simulink model "two"  (R2026a)
settings: Solver=VariableStepAuto
values from neighbouring files (symbols this model uses):
  L = 0.5    [MATLAB_6b.m]    (also in lab6_c.m)
  r = 0.1    [MATLAB_6b.m]    (also in lab6_c.m)
  WL = (V/r)-((L*Yr)/(2*r))    (= 20)    [MATLAB_6b.m]
  WR = (V/r)+((L*Yr)/(2*r))    (= 20)    [MATLAB_6b.m]
settings Model: Creator=m282256  LastModifiedBy=m282256

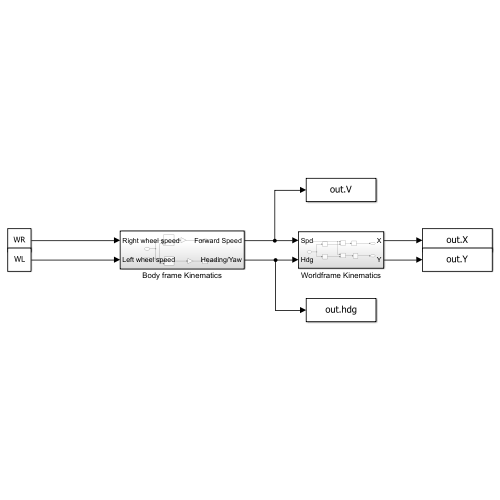
[thumbnail: Simulink's stored preview of the top-level diagram]
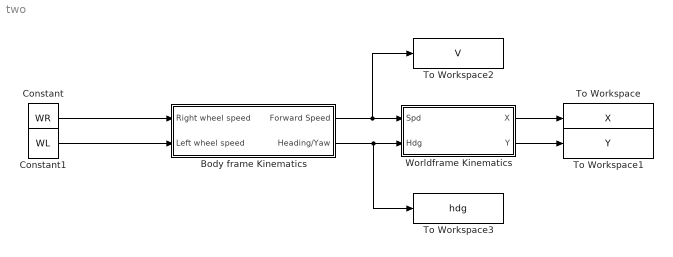
== system two ==
  Body frame Kinematics : Subsystem
  Constant : Constant  Value=WR
  Constant1 : Constant  Value=WL
  To Workspace : ToWorkspace  VariableName=X  SaveFormat=Timeseries  SampleTime=-1
  To Workspace1 : ToWorkspace  VariableName=Y  SaveFormat=Timeseries  SampleTime=-1
  To Workspace2 : ToWorkspace  VariableName=V  SaveFormat=Timeseries  SampleTime=-1
  To Workspace3 : ToWorkspace  VariableName=hdg  SaveFormat=Timeseries  SampleTime=-1
  Worldframe Kinematics : Subsystem
  wires:
  Constant1/1 -> Body frame Kinematics/2(Left wheel speed)
  Constant/1 -> Body frame Kinematics/1(Right wheel speed)
  Body frame Kinematics/2(Heading/Yaw) -> To Workspace3/1, Worldframe Kinematics/2(Hdg)
  Body frame Kinematics/1(Forward Speed) -> To Workspace2/1, Worldframe Kinematics/1(Spd)
  Worldframe Kinematics/2(Y) -> To Workspace1/1
  Worldframe Kinematics/1(X) -> To Workspace/1

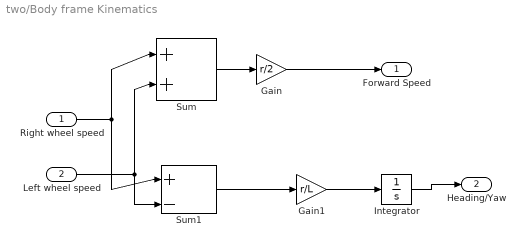
== system two/Body frame Kinematics ==
  Right wheel speed : Inport
  Left wheel speed : Inport  Port=2
  Gain : Gain  Gain=r/2
  Gain1 : Gain  Gain=r/L
  Integrator : Integrator
  Sum : Sum  Inputs=|++
  Sum1 : Sum  Inputs=|+-
  Forward Speed : Outport
  Heading/Yaw : Outport  Port=2
  wires:
  Right wheel speed/1 -> Sum/1, Sum1/1
  Sum1/1 -> Gain1/1
  Sum/1 -> Gain/1
  Left wheel speed/1 -> Sum/2, Sum1/2
  Gain1/1 -> Integrator/1
  Gain/1 -> Forward Speed/1
  Integrator/1 -> Heading/Yaw/1

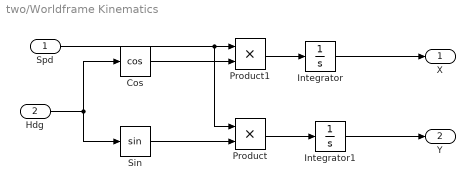
== system two/Worldframe Kinematics ==
  Spd : Inport
  Hdg : Inport  Port=2
  Cos : Trigonometry  Operator=cos
  Integrator : Integrator
  Integrator1 : Integrator
  Product : Product
  Product1 : Product
  Sin : Trigonometry
  X : Outport
  Y : Outport  Port=2
  wires:
  Spd/1 -> Product/1, Product1/1
  Hdg/1 -> Cos/1, Sin/1
  Cos/1 -> Product1/2
  Sin/1 -> Product/2
  Product/1 -> Integrator1/1
  Product1/1 -> Integrator/1
  Integrator/1 -> X/1
  Integrator1/1 -> Y/1
